simulink model "Icarus_Sim_recovered"  (R2026b)
settings: Solver=VariableStepAuto  StopTime=85  MaxStep=0.01
values from neighbouring files (symbols this model uses):
  A = pi * (d/2) ^ 2    (= 0.00754296396127)    [icarus_var.m]
  A_KF = [1 deltaT; 0 1]    [icarus_var.m]
  ADXL_Bias = 0.400*g    (= 3.924)    [icarus_var.m]
  ADXL_Range = 200*g    (= 1962)    [icarus_var.m]
  ADXL_Sample_Time = 1/ADXL_ODR_Hz    (= 0.00125)    [icarus_var.m]
  ADXL_Variance = ADXL_RMS_Noise^2    [icarus_var.m]
  Apogee_Drop = 1    [icarus_var.m]
  Arm_Alt = 100    [icarus_var.m]
  B_KF = [(0.5 * deltaT^2); deltaT]    [icarus_var.m]
  Backup_CoastTime = 11    [icarus_var.m]
  BNO_Accel_Bias = 0    [icarus_var.m]
  BNO_Accel_Range = 8*g    (= 78.48)    [icarus_var.m]
  BNO_Accel_Sample_Time = 1/BNO_Accel_Report_Rate    (= 0.002)    [icarus_var.m]
  BNO_Accel_Variance = BNO_Accel_Accuracy^2    (= 0.09)    [icarus_var.m]
  Boost_Trigger = 30    [icarus_var.m]
  Bump_Amp = 0    [icarus_var.m]
  Bump_Time = 1    [icarus_var.m]
  Bump_Width = 0.01    [icarus_var.m]
  C_KF = [1 0]    [icarus_var.m]
  Cd = 0.5    [icarus_var.m]
  CdA_drogue = (2 * m_dry * g) / (p0 * 25^2)    (= 0.0640646646395)    [icarus_var.m]
  CdA_main = (2 * m_dry * g) / (p0 * 6^2)    (= 1.1122337611)    [icarus_var.m]
  Coast_Trigger = 20    [icarus_var.m]
  deltaT = 0.01    [icarus_var.m]
  g = 9.81    [icarus_var.m]
  I_total = trapz(thrust_t, thrust_F)    [icarus_var.m]
  Ignition_Delay = 2    [icarus_var.m]
  L = 0.0065    [icarus_var.m]
  Landed_Trigger = 2    [icarus_var.m]
  Liftoff_Hold = 0.25    [icarus_var.m]
  m_dry = 2.5    [icarus_var.m]
  m_prop = 0.35    [icarus_var.m]
  Main_Trigger = 300    [icarus_var.m]
  P0 = 101325    [icarus_var.m]
  P_Abs_Accuracy = 75    [icarus_var.m]
  P_ODR_Sample_Time = 1/P_ODR_Hz    (= 0.0125)    [icarus_var.m]
  P_Variance = P_RMS_Noise^2    (= 0.0625)    [icarus_var.m]
  R = 287.05    [icarus_var.m]
  R_KF = P_Variance * (1/(p0*g))^2    (= 0.000432773966581)    [icarus_var.m]
  T0 = 288.15    [icarus_var.m]
  thrust_F = [0 300 250 230 180 0]    [icarus_var.m]
  thrust_t = [0 0.05 0.2 1.0 1.8 2.0]    [icarus_var.m]
  Timeout_Hold = 1    [icarus_var.m]
  Tolerance = 3    [icarus_var.m]
  Value_Hold = 0.05    [icarus_var.m]
undefined symbols (not defined in the file or in its folder): Discrete, Time
libraries: ctrlSharedLib x1
settings Model: Creator=Gene  LastModifiedBy=hdnat
settings SolverCC: AutoInsertRateTranBlk=on

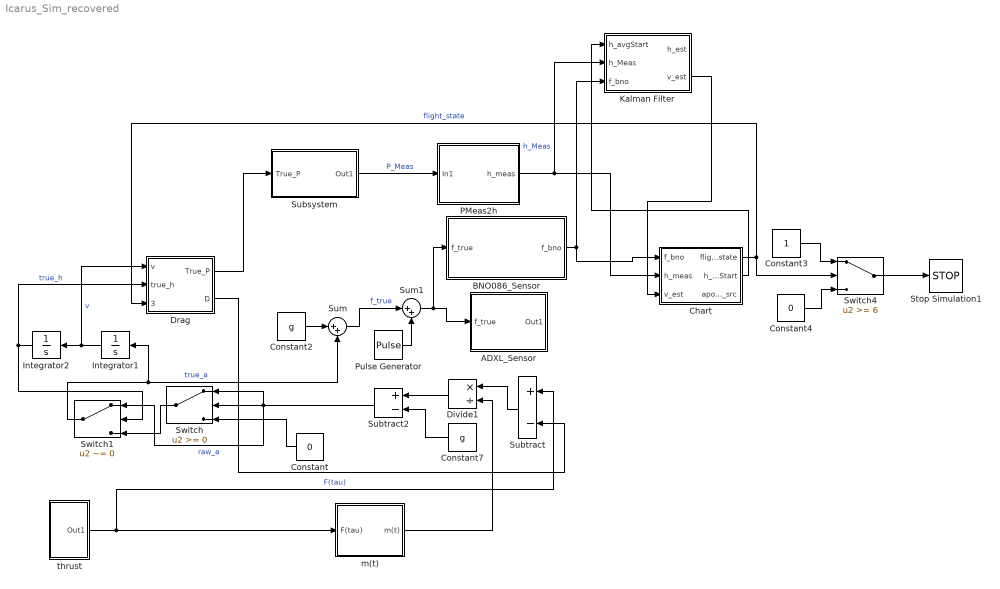
== system Icarus_Sim_recovered ==
  ADXL_Sensor : Subsystem
  BNO086_Sensor : Subsystem
  Chart : Stateflow chart  TreatAsAtomicUnit=on
  Constant : Constant  Value=0
  Constant2 : Constant  Value=g
  Constant3 : Constant
  Constant4 : Constant  Value=0
  Constant7 : Constant  Value=g
  Divide1 : Product  Inputs=*/
  Drag : Subsystem
  Integrator1 : Integrator
  Integrator2 : Integrator  LimitOutput=on  LowerSaturationLimit=0
  Kalman Filter : Subsystem
  PMeas2h : Subsystem
  Pulse Generator : DiscretePulseGenerator  PulseType=Time based  Amplitude=Bump_Amp  Period=1e4  PulseWidth=100 * Bump_Width/1e4  PhaseDelay=Bump_Time
  Stop Simulation1 : Stop
  Subsystem : Subsystem
  Subtract : Sum  Inputs=+-
  Subtract2 : Sum  Inputs=+-
  Sum : Sum  Inputs=|++
  Sum1 : Sum  Inputs=|++
  Switch : Switch  SaturateOnIntegerOverflow=off  InputSameDT=off
  Switch1 : Switch  Criteria=u2 ~= 0  SaturateOnIntegerOverflow=off  InputSameDT=off
  Switch4 : Switch  Threshold=6  SaturateOnIntegerOverflow=off  InputSameDT=off
  m(t) : Subsystem
  thrust : Subsystem
  wires:
  Integrator2/1 -> Drag/2(true_h), Switch1/2  "true_h"
  thrust/1(Out1) -> Subtract/1, m(t)/1(F(tau))  "F(tau)"
  Divide1/1 -> Subtract2/1
  Constant7/1 -> Subtract2/2
  Subtract2/1 -> Switch/1, Switch1/1, Switch/2  "raw_a"
  Subtract/1 -> Divide1/1
  Integrator1/1 -> Drag/1(v), Integrator2/1  "v"
  Constant/1 -> Switch/3
  Switch1/1 -> Sum/2, Integrator1/1  "true_a"
  Switch/1 -> Switch1/3
  Subsystem/1(Out1) -> PMeas2h/1(In1)  "P_Meas"
  PMeas2h/1(h_meas) -> Kalman Filter/2(h_Meas), Chart/2(h_meas)  "h_Meas"
  m(t)/1(m(t)) -> Divide1/2
  Drag/1(True_P) -> Subsystem/1(True_P)
  Drag/2(D) -> Subtract/2
  Constant2/1 -> Sum/1
  Sum/1 -> Sum1/1  "f_true"
  BNO086_Sensor/1(f_bno) -> Chart/1(f_bno), Kalman Filter/3(f_bno)
  Chart/1(flight_state) -> Switch4/2, Drag/3(flight_state)  "flight_state"
  Switch4/1 -> Stop Simulation1/1
  Constant3/1 -> Switch4/1
  Constant4/1 -> Switch4/3
  Chart/2(h_avgStart) -> Kalman Filter/1(h_avgStart)
  Kalman Filter/2(v_est) -> Chart/3(v_est)
  Pulse Generator/1 -> Sum1/2
  Sum1/1 -> BNO086_Sensor/1(f_true), ADXL_Sensor/1(f_true)

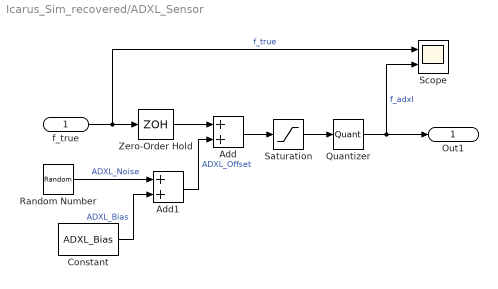
== system Icarus_Sim_recovered/ADXL_Sensor ==
  f_true : Inport
  Add : Sum
  Add1 : Sum
  Constant : Constant  Value=ADXL_Bias
  Quantizer : Quantizer  QuantizationInterval=ADXL_LSB_Size
  Random Number : RandomNumber  Variance=ADXL_Variance  Seed=100  SampleTime=0.01
  Saturation : Saturate  UpperLimit=ADXL_Range  LowerLimit=-ADXL_Range
  Scope : Scope  NumInputPorts=2
      settings: ActiveDisplayYMinimum=-30.113183434671704  ActiveDisplayYMaximum=125.12070927051909  DataLoggingVariableName=ScopeData3
  Zero-Order Hold : ZeroOrderHold  SampleTime=ADXL_Sample_Time
  Out1 : Outport
  wires:
  f_true/1 -> Scope/1, Zero-Order Hold/1  "f_true"
  Zero-Order Hold/1 -> Add/1
  Random Number/1 -> Add1/1  "ADXL_Noise"
  Constant/1 -> Add1/2  "ADXL_Bias"
  Add1/1 -> Add/2  "ADXL_Offset"
  Add/1 -> Saturation/1
  Saturation/1 -> Quantizer/1
  Quantizer/1 -> Scope/2, Out1/1  "f_adxl"

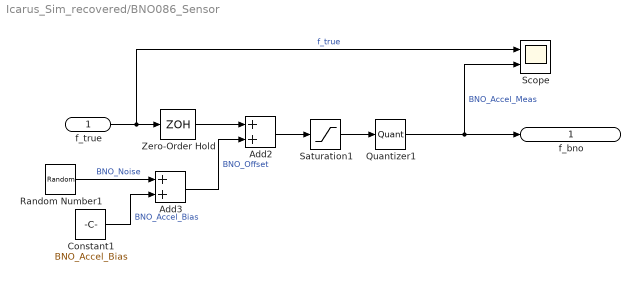
== system Icarus_Sim_recovered/BNO086_Sensor ==
  f_true : Inport
  Add2 : Sum
  Add3 : Sum
  Constant1 : Constant  Value=BNO_Accel_Bias
  Quantizer1 : Quantizer  QuantizationInterval=BNO_Accel_LSB
  Random Number1 : RandomNumber  Variance=BNO_Accel_Variance  Seed=50  SampleTime=0.01
  Saturation1 : Saturate  UpperLimit=BNO_Accel_Range  LowerLimit=-BNO_Accel_Range
  Scope : Scope  NumInputPorts=2
      settings: ActiveDisplayYMinimum=-30.065542476173064  ActiveDisplayYMaximum=120.55081978555759  DataLoggingVariableName=ScopeData4
  Zero-Order Hold : ZeroOrderHold  SampleTime=BNO_Accel_Sample_Time
  f_bno : Outport
  wires:
  f_true/1 -> Scope/1, Zero-Order Hold/1  "f_true"
  Add3/1 -> Add2/2  "BNO_Offset"
  Zero-Order Hold/1 -> Add2/1
  Random Number1/1 -> Add3/1  "BNO_Noise"
  Constant1/1 -> Add3/2  "BNO_Accel_Bias"
  Add2/1 -> Saturation1/1
  Saturation1/1 -> Quantizer1/1
  Quantizer1/1 -> Scope/2, f_bno/1  "BNO_Accel_Meas"

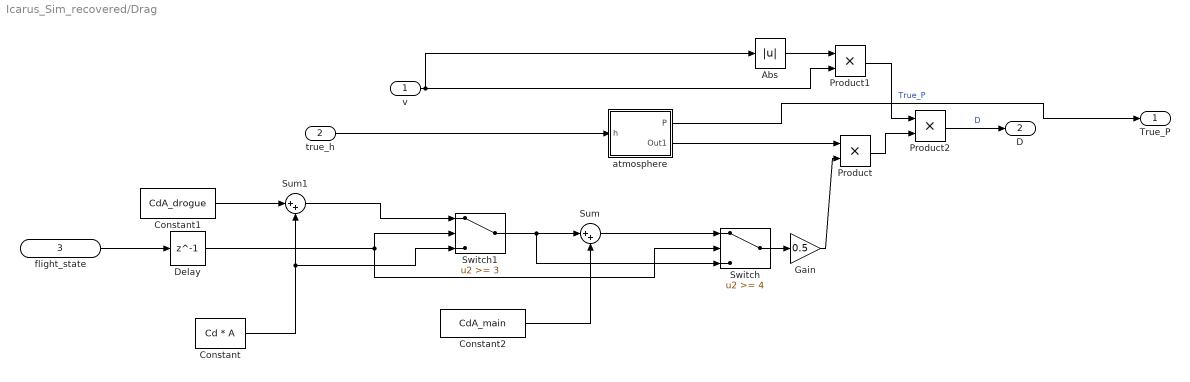
== system Icarus_Sim_recovered/Drag ==
  v : Inport
  true_h : Inport  Port=2
  flight_state : Inport  Port=3
  Abs : Abs  SaturateOnIntegerOverflow=off
  Constant : Constant  Value=Cd * A
  Constant1 : Constant  Value=CdA_drogue
  Constant2 : Constant  Value=CdA_main
  Delay : Delay  DelayLength=1
  Gain : Gain  Gain=0.5
  Product : Product
  Product1 : Product
  Product2 : Product
  Sum : Sum  Inputs=|++
  Sum1 : Sum  Inputs=|++
  Switch : Switch  Threshold=4  SaturateOnIntegerOverflow=off  InputSameDT=off
  Switch1 : Switch  Threshold=3  SaturateOnIntegerOverflow=off  InputSameDT=off
  atmosphere : Subsystem
  True_P : Outport
  D : Outport  Port=2
  wires:
  Product1/1 -> Product2/1
  Product/1 -> Product2/2
  atmosphere/2(Out1) -> Product/1
  Abs/1 -> Product1/1
  true_h/1 -> atmosphere/1(h)
  v/1 -> Abs/1, Product1/2
  atmosphere/1(P) -> True_P/1  "True_P"
  Product2/1 -> D/1  "D"
  Sum/1 -> Switch/1
  Switch1/1 -> Switch/3, Sum/1
  Sum1/1 -> Switch1/1
  Constant1/1 -> Sum1/1
  Constant/1 -> Switch1/3, Sum1/2
  Constant2/1 -> Sum/2
  Gain/1 -> Product/2
  Switch/1 -> Gain/1
  flight_state/1 -> Delay/1
  Delay/1 -> Switch/2, Switch1/2

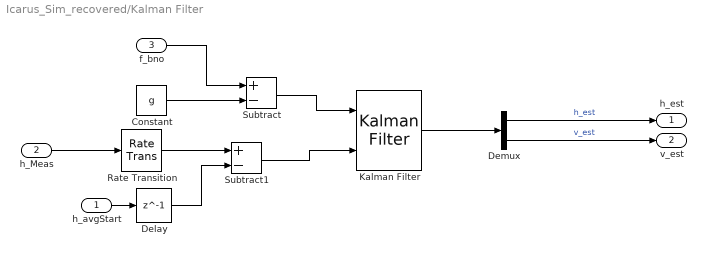
== system Icarus_Sim_recovered/Kalman Filter ==
  h_avgStart : Inport
  h_Meas : Inport  Port=2
  f_bno : Inport  Port=3
  Constant : Constant  Value=g
  Delay : Delay  DelayLength=1  SampleTime=deltaT
  Demux : Demux  Outputs=2
  Kalman Filter : ctrlSharedLib/Kalman Filter  TimeDomain=Discrete-Time  UseCurrentEstimator=on  ModelSource=Individual A, B, C, D matrices  ModelSourceVariable=ss(0.95,1,1,0,1)  A=A_KF  B=B_KF  C=C_KF  D=0  NumberOfStates=1  NumberOfInputs=1  NumberOfOutputs=1  Ts=deltaT  InitialEstimateSource=Dialog  X0=[0; 0]  P0=diag([1, 1])  UseK=off  UseGH=off  G=1  TimeInvariantG=on  H=0  TimeInvariantH=on  NumberOfProcessNoiseInputs=1  Q=Q_KF  TimeInvariantQ=on  R=R_KF  TimeInvariantR=on  N=0  TimeInvariantN=on  AddInputPort=on  AddEnablePort=off  OutputEstimatedY=off  OutputP=off
  Rate Transition : RateTransition  Deterministic=off  OutPortSampleTime=deltaT
  Subtract : Sum  Inputs=+-
  Subtract1 : Sum  Inputs=+-
  h_est : Outport
  v_est : Outport  Port=2
  wires:
  Kalman Filter/1 -> Demux/1
  Demux/2 -> v_est/1  "v_est"
  Demux/1 -> h_est/1  "h_est"
  f_bno/1 -> Subtract/1
  Constant/1 -> Subtract/2
  Subtract/1 -> Kalman Filter/1
  Subtract1/1 -> Kalman Filter/2
  h_avgStart/1 -> Delay/1
  Delay/1 -> Subtract1/2
  Rate Transition/1 -> Subtract1/1
  h_Meas/1 -> Rate Transition/1

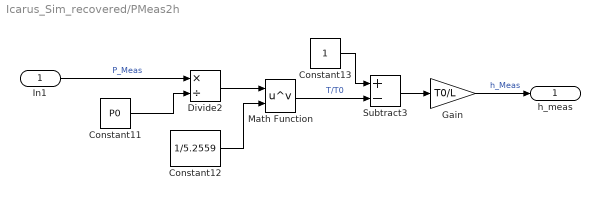
== system Icarus_Sim_recovered/PMeas2h ==
  In1 : Inport
  Constant11 : Constant  Value=P0
  Constant12 : Constant  Value=1/5.2559
  Constant13 : Constant
  Divide2 : Product  Inputs=*/
  Gain : Gain  Gain=T0/L
  Math Function : Math  Operator=pow
  Subtract3 : Sum  Inputs=+-
  h_meas : Outport
  wires:
  Constant13/1 -> Subtract3/1
  Math Function/1 -> Subtract3/2  "T/T0"
  In1/1 -> Divide2/1  "P_Meas"
  Gain/1 -> h_meas/1  "h_Meas"
  Subtract3/1 -> Gain/1
  Constant11/1 -> Divide2/2
  Divide2/1 -> Math Function/1
  Constant12/1 -> Math Function/2

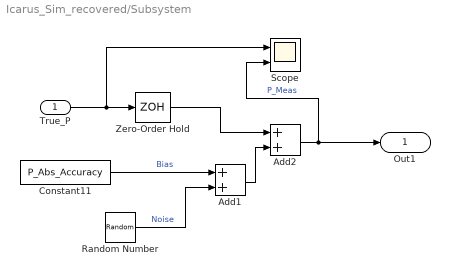
== system Icarus_Sim_recovered/Subsystem ==
  True_P : Inport
  Add1 : Sum
  Add2 : Sum
  Constant11 : Constant  Value=P_Abs_Accuracy
  Random Number : RandomNumber  Variance=P_Variance  Seed=69  SampleTime=0.01
  Scope : Scope  NumInputPorts=2
      settings: ActiveDisplayYMinimum=101303.95900046229  ActiveDisplayYMaximum=101452.80556619991
  Zero-Order Hold : ZeroOrderHold  SampleTime=P_ODR_Sample_Time
  Out1 : Outport
  wires:
  Constant11/1 -> Add1/1  "Bias"
  Random Number/1 -> Add1/2  "Noise"
  Add1/1 -> Add2/2
  True_P/1 -> Scope/1, Zero-Order Hold/1
  Add2/1 -> Scope/2, Out1/1  "P_Meas"
  Zero-Order Hold/1 -> Add2/1

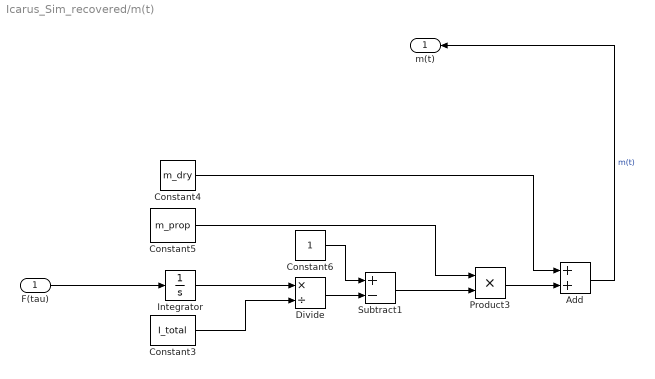
== system Icarus_Sim_recovered/m(t) ==
  F(tau) : Inport
  Add : Sum
  Constant3 : Constant  Value=I_total
  Constant4 : Constant  Value=m_dry
  Constant5 : Constant  Value=m_prop
  Constant6 : Constant
  Divide : Product  Inputs=*/
  Integrator : Integrator
  Product3 : Product
  Subtract1 : Sum  Inputs=+-
  m(t) : Outport
  wires:
  Divide/1 -> Subtract1/2
  Constant5/1 -> Product3/1
  Add/1 -> m(t)/1  "m(t)"
  Constant4/1 -> Add/1
  Constant6/1 -> Subtract1/1
  Subtract1/1 -> Product3/2
  Integrator/1 -> Divide/1
  Product3/1 -> Add/2
  F(tau)/1 -> Integrator/1
  Constant3/1 -> Divide/2

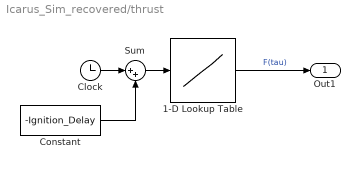
== system Icarus_Sim_recovered/thrust ==
  1-D Lookup Table : Lookup_n-D  NumberOfTableDimensions=1  BreakpointsForDimension1=thrust_t  Table=thrust_F  ExtrapMethod=Clip  InternalRulePriority=Speed  RndMeth=Simplest
  Clock : Clock
  Constant : Constant  Value=-Ignition_Delay
  Sum : Sum  Inputs=|++
  Out1 : Outport
  wires:
  1-D Lookup Table/1 -> Out1/1  "F(tau)"
  Clock/1 -> Sum/1
  Sum/1 -> 1-D Lookup Table/1
  Constant/1 -> Sum/2

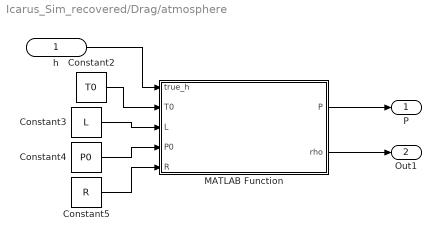
== system Icarus_Sim_recovered/Drag/atmosphere ==
  h : Inport
  Constant2 : Constant  Value=T0
  Constant3 : Constant  Value=L
  Constant4 : Constant  Value=P0
  Constant5 : Constant  Value=R
  MATLAB Function : MATLAB Function  TreatAsAtomicUnit=on
  P : Outport
  Out1 : Outport  Port=2
  wires:
  Constant2/1 -> MATLAB Function/2(T0)
  MATLAB Function/1(P) -> P/1
  h/1 -> MATLAB Function/1(true_h)
  Constant3/1 -> MATLAB Function/3(L)
  Constant4/1 -> MATLAB Function/4(P0)
  MATLAB Function/2(rho) -> Out1/1
  Constant5/1 -> MATLAB Function/5(R)

== matlab function Icarus_Sim_recovered/Drag/atmosphere/MATLAB Function ==
  data: true_h input; P output; T0 input; L input; P0 input; R input; rho output
function [P, rho] = atmosphere (true_h, T0, L, P0, R)
    T = T0 - L * true_h; %temperature at altitude
    P = P0 * (T/T0)^5.2559 %Pressure Pa
    rho = P / (R * T); %air density
end

== stateflow chart Icarus_Sim_recovered/Chart ==
  settings: updateMethod=DISCRETE  sampleTime=0.01
  state Pad
    entry:
    flight_state = 0;
    h_sum = 0;
    h_sumCount = 0;
    h_avgStart = 0;
    apogee_src = 0;
    during:
    h_sum = h_sum + h_meas;
    h_sumCount = h_sumCount + 1;
    h_avgStart = h_sum/h_sumCount;
    exit:
    h_avgStart = h_sum/h_sumCount;
  state Boost
    entry:
    flight_state = 1;
  state Coast
    entry:
    flight_state = 2;
    maxH = h_meas;
    during:
    maxH = max(maxH, h_meas);
  state Main
    entry:
    flight_state = 4;
    h_ref = h_meas;
    during:
    if abs(h_ref - h_meas) > Tolerance
    h_ref = h_meas;
    end
  state Apogee
    entry:
    flight_state = 3;
  state End
    entry:
    flight_state = 6;
  state Landed
    entry:
    flight_state = 5;
  (default) -> Pad
  Coast -> Apogee [order 3] : [after(Backup_CoastTime, sec) && (h_meas - h_avgStart >= Arm_Alt)]{apogee_src = 3;}
  Pad -> Boost : [duration(f_bno>=Boost_Trigger) >=Liftoff_Hold]
  Boost -> Coast : [duration(f_bno<=Coast_Trigger) >= Value_Hold]
  Coast -> Apogee [order 2] : [((duration(maxH - h_meas > Apogee_Drop) >= Timeout_Hold) || (duration(v_est <= 0) >=Timeout_Hold)) && (h_meas - h_avgStart >= Arm_Alt)]{apogee_src = 2;}
  Coast -> Apogee [order 1] : [(duration(maxH - h_meas > Apogee_Drop) >= Value_Hold) && (duration(v_est <= 0) >=Value_Hold) && (h_meas - h_avgStart >= Arm_Alt)]{apogee_src = 1;}
  Apogee -> Main : [duration(h_meas - h_avgStart <= Main_Trigger) >= Value_Hold]
  Landed -> End : [duration(flight_state == 5) >= 2]
  Main -> Landed : [duration(abs(h_ref - h_meas) <= Tolerance) >= Landed_Trigger]
  data: f_bno input; flight_state output =0; h_meas input; maxH local =0; Apogee_Drop parameter double; h_sum local =0; h_sumCount local =0; Value_Hold parameter double; Boost_Trigger parameter double; Coast_Trigger parameter double; Main_Trigger parameter double; h_ref local =0; Tolerance parameter double; Landed_Trigger parameter double; h_avgStart output =0; v_est input; Timeout_Hold parameter; Backup_CoastTime parameter; apogee_src output =0; Liftoff_Hold parameter; Arm_Alt parameter
